simulink model "lorenz3d"  (Simulink 8.4)
settings: Solver=ode45  SolverMode=SingleTasking  StartTime=0.0  StopTime=Inf  RelTol=1e-3
undefined symbols (not defined in the file or in its folder): sfun3d
settings Model: Creator=The MathWorks Inc.  LastModifiedBy=gcampa  ExtModeTrigMode=oneshot  ExtModeArmWhenConnect=off
settings DataIOCC: SignalLoggingSaveFormat=Dataset
settings OptimizationCC: BlockReduction=off  BooleanDataType=off  ExpressionDepthLimit=128
settings DebuggingCC: SaveWithParameterizedLinksMsg=none  SignalResolutionControl=TryResolveAllWithWarning  SolverPrmCheckMsg=none  FcnCallInpInsideContextMsg=EnableAllAsError  StateNameClashWarn=none
settings HardwareCC: TargetUnknown=on
settings GRTTargetCC: CombineOutputUpdateFcns=on  GRTInterface=off

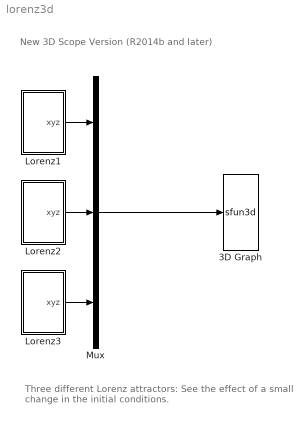
== system lorenz3d ==
  note: Three different Lorenz attractors:
      | See the effect of a small change in the initial conditions.
  note: New 3D Scope Version (R2014b and later)
  3D Graph : S-Function  LoadFcn=sfun3d([],[],[],'LoadBlock')  StartFcn=sfun3d([],[],[],'Start')  StopFcn=sfun3d([],[],[],'Stop')  FunctionName=sfun3d  Parameters=ax,T,np,cp,gd,ls,mk  EnableBusSupport=off  mask(3D Graph){np=3, ax=[-30 30 -20 30 0 50], cp=[1 1 20], gd=on, ls=-, mk=none, T=0.01}
      mask prompts: np "Number of point (lines)"; ax "[xmin xmax  ymin ymax zmin zmax]"; cp "Camera position (use [0 0 1] for 2D XY view)"; gd "Grid (on|off)"; ls "LineStyle"; mk "Marker"; T "Sampling Time"
      mask help:
      | This block plots the position of several points in the XYZ space. The input contains the coordinates of all the points (x1,y1,z1,x2,y2,z2,...).
      | The number of points (lines), the XYZ ranges, camera position, grid, linestyle, marker and sampling time, can be set as mask parameters.
      settings: CopyFcn=sfun3d([],[],[],'CopyBlock')  DeleteFcn=sfun3d([],[],[],'DeleteBlock')  NameChangeFcn=sfun3d([],[],[],'NameChange')
      mask Help:
      | This block plots the position of several points in the XYZ space. The input contains the coordinates of all the points (x1,y1,z1,x2,y2,z2,...).
      | The number of points (lines), the XYZ ranges, camera position, grid, linestyle, marker and sampling time, can be set as mask parameters.
      mask TypeOptions ls: - | -- | : | -. | none
      mask TypeOptions mk: none | . | + | o | * | x | square | diamond | v | ^ | > | < | pentagram | hexagram
      mask Display: plot([.05 .95 .95 .05 .05],[.45 .45 .95 .95 .45], 0.5+cos(0:0.1:2*pi)*0.3,0.7+sin(0:0.1:2*pi)*0.2)
  Lorenz1 : Subsystem  mask(Lorenz Attractor System){s=10, r=28, b=2+2/3, xyz0=[1 1 1]}
      mask prompts: s "sigma"; r "rho"; b "beta"; xyz0 "Initial State (x0, y0, y0)"
      mask help:
      | This autonomous system generates the lorentz attractor:
      | xdot=sigma*(x-y); ydot=rho*x-y-x*z; zdot=-beta*z+x*y;
      | Parameters and initial state can be selected from the mask.
      mask Help:
      | This autonomous system generates the lorentz attractor.
      | Parameters and initial state can be selected from the mask.
      | <p>
      | The system equations are:
      | xdot = sigma*(x-y),
      | ydot = rho*x-y-x*z,
      | zdot = -beta*z+x*y,
  Lorenz2 : Subsystem  mask(Lorenz Attractor System){s=10, r=28, b=2+2/3, xyz0=[2 2 2]}
      mask prompts: s "sigma"; r "rho"; b "beta"; xyz0 "Initial State (x0, y0, y0)"
      mask help:
      | This autonomous system generates the lorentz attractor:
      | xdot=sigma*(x-y); ydot=rho*x-y-x*z; zdot=-beta*z+x*y;
      | Parameters and initial state can be selected from the mask.
      mask Help:
      | This autonomous system generates the lorentz attractor.
      | Parameters and initial state can be selected from the mask.
      | <p>
      | The system equations are:
      | xdot = sigma*(x-y),
      | ydot = rho*x-y-x*z,
      | zdot = -beta*z+x*y,
  Lorenz3 : Subsystem  mask(Lorenz Attractor System){s=10, r=28, b=2+2/3, xyz0=[3 3 3]}
      mask prompts: s "sigma"; r "rho"; b "beta"; xyz0 "Initial State (x0, y0, y0)"
      mask help:
      | This autonomous system generates the lorentz attractor:
      | xdot=sigma*(x-y); ydot=rho*x-y-x*z; zdot=-beta*z+x*y;
      | Parameters and initial state can be selected from the mask.
      mask Help:
      | This autonomous system generates the lorentz attractor.
      | Parameters and initial state can be selected from the mask.
      | <p>
      | The system equations are:
      | xdot = sigma*(x-y),
      | ydot = rho*x-y-x*z,
      | zdot = -beta*z+x*y,
  Mux : Mux  Inputs=[3 3 3]
  wires:
  Lorenz1/1(xyz) -> Mux/1
  Lorenz2/1(xyz) -> Mux/2
  Lorenz3/1(xyz) -> Mux/3
  Mux/1 -> 3D Graph/1

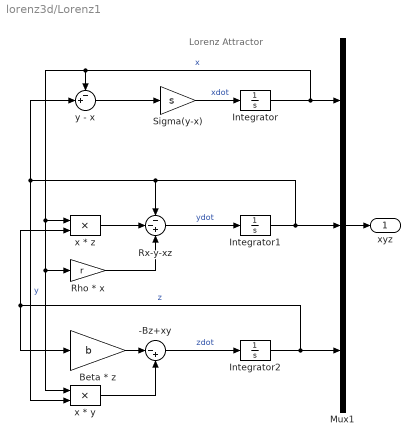
== system lorenz3d/Lorenz1 ==
  note: Lorenz Attractor
  -Bz+xy : Sum  Inputs=|-+  SaturateOnIntegerOverflow=on  InputSameDT=on  OutDataTypeStr=Inherit: Same as first input
  Beta * z : Gain  Gain=b  SaturateOnIntegerOverflow=on  OutDataTypeStr=Inherit: Same as input  ParamDataTypeStr=Inherit: Same as input
  Integrator : Integrator  InitialCondition=xyz0(1)
  Integrator1 : Integrator  InitialCondition=xyz0(2)
  Integrator2 : Integrator  InitialCondition=xyz0(3)
  Mux1 : Mux  Inputs=3
  Rho * x : Gain  Gain=r  SaturateOnIntegerOverflow=on  OutDataTypeStr=Inherit: Same as input  ParamDataTypeStr=Inherit: Same as input
  Rx-y-xz : Sum  Inputs=--+  SaturateOnIntegerOverflow=on  InputSameDT=on  OutDataTypeStr=Inherit: Same as first input
  Sigma(y-x) : Gain  Gain=s  SaturateOnIntegerOverflow=on  OutDataTypeStr=Inherit: Same as input  ParamDataTypeStr=Inherit: Same as input
  x * y : Product  SaturateOnIntegerOverflow=on  RndMeth=Zero  InputSameDT=on  OutDataTypeStr=Inherit: Same as first input
  x * z : Product  SaturateOnIntegerOverflow=on  RndMeth=Zero  InputSameDT=on  OutDataTypeStr=Inherit: Same as first input
  y - x : Sum  Inputs=-+|  SaturateOnIntegerOverflow=on  InputSameDT=on  OutDataTypeStr=Inherit: Same as first input
  xyz : Outport
  wires:
  Sigma(y-x)/1 -> Integrator/1  "xdot"
  y - x/1 -> Sigma(y-x)/1
  Rx-y-xz/1 -> Integrator1/1  "ydot"
  x * z/1 -> Rx-y-xz/2
  Integrator2/1 -> x * z/2, Beta * z/1, Mux1/3  "z"
  Integrator1/1 -> Rx-y-xz/1, y - x/2, x * y/2, Mux1/2  "y"
  Integrator/1 -> y - x/1, x * z/1, Rho * x/1, x * y/1, Mux1/1  "x"
  -Bz+xy/1 -> Integrator2/1  "zdot"
  Beta * z/1 -> -Bz+xy/1
  x * y/1 -> -Bz+xy/2
  Mux1/1 -> xyz/1
  Rho * x/1 -> Rx-y-xz/3

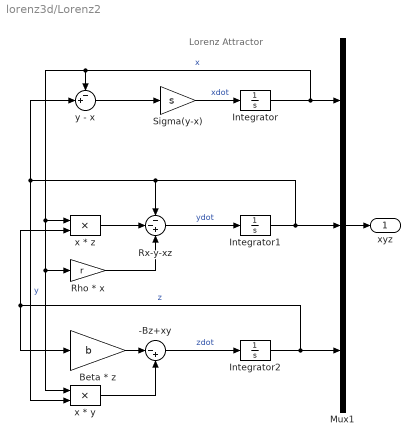
== system lorenz3d/Lorenz2 ==
  note: Lorenz Attractor
  -Bz+xy : Sum  Inputs=|-+  SaturateOnIntegerOverflow=on  InputSameDT=on  OutDataTypeStr=Inherit: Same as first input
  Beta * z : Gain  Gain=b  SaturateOnIntegerOverflow=on  OutDataTypeStr=Inherit: Same as input  ParamDataTypeStr=Inherit: Same as input
  Integrator : Integrator  InitialCondition=xyz0(1)
  Integrator1 : Integrator  InitialCondition=xyz0(2)
  Integrator2 : Integrator  InitialCondition=xyz0(3)
  Mux1 : Mux  Inputs=3
  Rho * x : Gain  Gain=r  SaturateOnIntegerOverflow=on  OutDataTypeStr=Inherit: Same as input  ParamDataTypeStr=Inherit: Same as input
  Rx-y-xz : Sum  Inputs=--+  SaturateOnIntegerOverflow=on  InputSameDT=on  OutDataTypeStr=Inherit: Same as first input
  Sigma(y-x) : Gain  Gain=s  SaturateOnIntegerOverflow=on  OutDataTypeStr=Inherit: Same as input  ParamDataTypeStr=Inherit: Same as input
  x * y : Product  SaturateOnIntegerOverflow=on  RndMeth=Zero  InputSameDT=on  OutDataTypeStr=Inherit: Same as first input
  x * z : Product  SaturateOnIntegerOverflow=on  RndMeth=Zero  InputSameDT=on  OutDataTypeStr=Inherit: Same as first input
  y - x : Sum  Inputs=-+|  SaturateOnIntegerOverflow=on  InputSameDT=on  OutDataTypeStr=Inherit: Same as first input
  xyz : Outport
  wires:
  Mux1/1 -> xyz/1
  x * y/1 -> -Bz+xy/2
  Beta * z/1 -> -Bz+xy/1
  -Bz+xy/1 -> Integrator2/1  "zdot"
  Integrator/1 -> Mux1/1, x * y/1, Rho * x/1, x * z/1, y - x/1  "x"
  Integrator1/1 -> Mux1/2, x * y/2, y - x/2, Rx-y-xz/1  "y"
  Integrator2/1 -> Mux1/3, Beta * z/1, x * z/2  "z"
  x * z/1 -> Rx-y-xz/2
  Rx-y-xz/1 -> Integrator1/1  "ydot"
  y - x/1 -> Sigma(y-x)/1
  Sigma(y-x)/1 -> Integrator/1  "xdot"
  Rho * x/1 -> Rx-y-xz/3

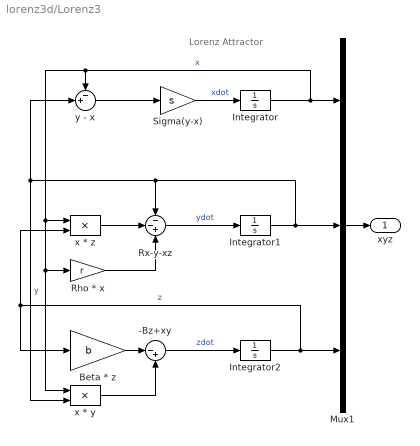
== system lorenz3d/Lorenz3 ==
  note: Lorenz Attractor
  -Bz+xy : Sum  Inputs=|-+  SaturateOnIntegerOverflow=on  InputSameDT=on  OutDataTypeStr=Inherit: Same as first input
  Beta * z : Gain  Gain=b  SaturateOnIntegerOverflow=on  OutDataTypeStr=Inherit: Same as input  ParamDataTypeStr=Inherit: Same as input
  Integrator : Integrator  InitialCondition=xyz0(1)
  Integrator1 : Integrator  InitialCondition=xyz0(2)
  Integrator2 : Integrator  InitialCondition=xyz0(3)
  Mux1 : Mux  Inputs=3
  Rho * x : Gain  Gain=r  SaturateOnIntegerOverflow=on  OutDataTypeStr=Inherit: Same as input  ParamDataTypeStr=Inherit: Same as input
  Rx-y-xz : Sum  Inputs=--+  SaturateOnIntegerOverflow=on  InputSameDT=on  OutDataTypeStr=Inherit: Same as first input
  Sigma(y-x) : Gain  Gain=s  SaturateOnIntegerOverflow=on  OutDataTypeStr=Inherit: Same as input  ParamDataTypeStr=Inherit: Same as input
  x * y : Product  SaturateOnIntegerOverflow=on  RndMeth=Zero  InputSameDT=on  OutDataTypeStr=Inherit: Same as first input
  x * z : Product  SaturateOnIntegerOverflow=on  RndMeth=Zero  InputSameDT=on  OutDataTypeStr=Inherit: Same as first input
  y - x : Sum  Inputs=-+|  SaturateOnIntegerOverflow=on  InputSameDT=on  OutDataTypeStr=Inherit: Same as first input
  xyz : Outport
  wires:
  Sigma(y-x)/1 -> Integrator/1  "xdot"
  y - x/1 -> Sigma(y-x)/1
  Rx-y-xz/1 -> Integrator1/1  "ydot"
  x * z/1 -> Rx-y-xz/2
  Integrator2/1 -> x * z/2, Beta * z/1, Mux1/3  "z"
  Integrator1/1 -> Rx-y-xz/1, y - x/2, x * y/2, Mux1/2  "y"
  Integrator/1 -> y - x/1, x * z/1, Rho * x/1, x * y/1, Mux1/1  "x"
  -Bz+xy/1 -> Integrator2/1  "zdot"
  Beta * z/1 -> -Bz+xy/1
  x * y/1 -> -Bz+xy/2
  Mux1/1 -> xyz/1
  Rho * x/1 -> Rx-y-xz/3
